simulink model "DSC4to1Diodes"  (R2022a)
settings: Solver=VariableStepAuto  StartTime=0.0  StopTime=10.0  RelTol=1e-3
undefined symbols (not defined in the file): plecs
settings Model: Creator=dcostine  LastModifiedBy=dcostine
settings DebuggingCC: UnconnectedInputMsg=warning  UnconnectedOutputMsg=warning  UnconnectedLineMsg=warning
settings RTWCC: DLArmComputeVersion=19.05

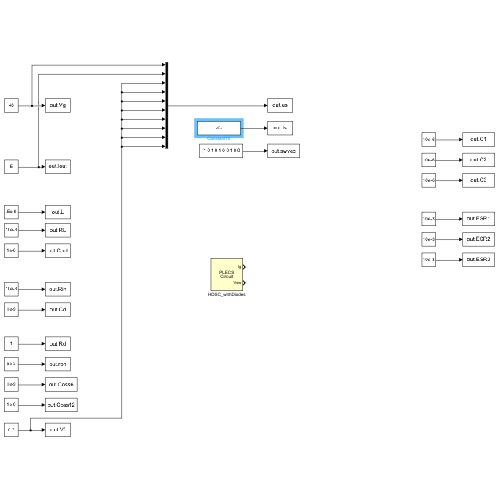
[thumbnail: Simulink's stored preview of the top-level diagram]
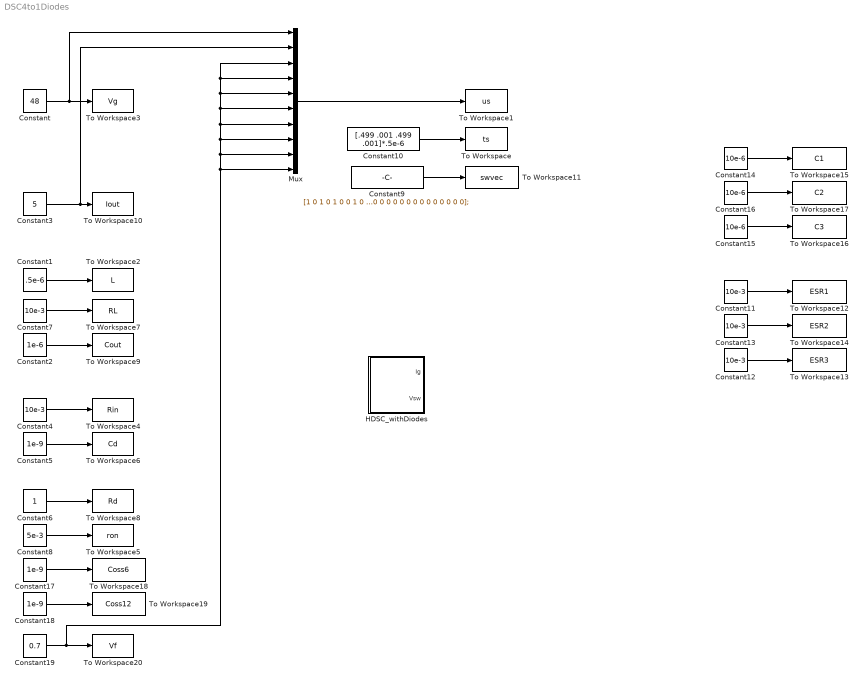
== system DSC4to1Diodes ==
  Constant : Constant  Value=48
  Constant1 : Constant  Value=.5e-6
  Constant10 : Constant  Value=[.499 .001 .499 .001]*.5e-6
  Constant{4,7,11..13} (5 alike) : Constant  Value=10e-3
  Constant14 : Constant  Value=10e-6
  Constant15 : Constant  Value=10e-6
  Constant16 : Constant  Value=10e-6
  Constant17 : Constant  Value=1e-9
  Constant18 : Constant  Value=1e-9
  Constant19 : Constant  Value=0.7
  Constant2 : Constant  Value=1e-6
  Constant3 : Constant  Value=5
  Constant5 : Constant  Value=1e-9
  Constant6 : Constant
  Constant8 : Constant  Value=5e-3
  Constant9 : Constant  Value=[1 0 1 0 1 0 0 1 0 0 0 0 0 0 0 0; 0 0 0 0 0 0 0 0 0 0 0 0 0 0 0 0; 0 1 0 1 0 1 1 0 0 0 0 0 0 0 0 0; 0 0 0 0 0 0 0 0 0 0 0 0 0 0 0 0];
  HDSC_withDiodes : Subsystem  LoadFcn=plecs('sl', 200);  InitFcn=plecs('sl', 214);  StartFcn=plecs('sl', 208);  StopFcn=plecs('sl', 209);  mask(PlecsCircuit){PLECSData=<binary blob, 3580 chars, not shown>}
      mask prompts: PLECSData "PLECS Data (Do not delete or modify!)"
      mask init:
      | % PLACE CUSTOM INITIALIZATIONS ABOVE
      | % DO NOT REMOVE
      | plecs('sl', 215);
      | % DO NOT REMOVE
      settings: CopyFcn=plecs('sl', 203);  DeleteFcn=plecs('sl', 205);  UndoDeleteFcn=plecs('sl', 206);  PreSaveFcn=plecs('sl', 211);  PostSaveFcn=plecs('sl', 201);  NameChangeFcn=plecs('sl', 210);  DestroyFcn=plecs('sl', 207);  PreCopyFcn=plecs('sl', 216);  OpenFcn=plecs('sl', 202);  ErrorFcn=plerrorfcn
      mask Help: web(['file:///' fullfile(plecsdoc, 'creatingacircuit.html')])
      mask Display: disp('PLECS\nCircuit')
  Mux : Mux  Inputs=10
  To Workspace : ToWorkspace  VariableName=ts  SampleTime=-1
  To Workspace1 : ToWorkspace  VariableName=us  SampleTime=-1
  To Workspace10 : ToWorkspace  VariableName=Iout  SampleTime=-1
  To Workspace11 : ToWorkspace  VariableName=swvec  SampleTime=-1
  To Workspace12 : ToWorkspace  VariableName=ESR1  SampleTime=-1
  To Workspace13 : ToWorkspace  VariableName=ESR3  SampleTime=-1
  To Workspace14 : ToWorkspace  VariableName=ESR2  SampleTime=-1
  To Workspace15 : ToWorkspace  VariableName=C1  SampleTime=-1
  To Workspace16 : ToWorkspace  VariableName=C3  SampleTime=-1
  To Workspace17 : ToWorkspace  VariableName=C2  SampleTime=-1
  To Workspace18 : ToWorkspace  VariableName=Coss6  SampleTime=-1
  To Workspace19 : ToWorkspace  VariableName=Coss12  SampleTime=-1
  To Workspace2 : ToWorkspace  VariableName=L  SampleTime=-1
  To Workspace20 : ToWorkspace  VariableName=Vf  SampleTime=-1
  To Workspace3 : ToWorkspace  VariableName=Vg  SampleTime=-1
  To Workspace4 : ToWorkspace  VariableName=Rin  SampleTime=-1
  To Workspace5 : ToWorkspace  VariableName=ron  SampleTime=-1
  To Workspace6 : ToWorkspace  VariableName=Cd  SampleTime=-1
  To Workspace7 : ToWorkspace  VariableName=RL  SampleTime=-1
  To Workspace8 : ToWorkspace  VariableName=Rd  SampleTime=-1
  To Workspace9 : ToWorkspace  VariableName=Cout  SampleTime=-1
  wires:
  Mux/1 -> To Workspace1/1
  Constant1/1 -> To Workspace2/1
  Constant/1 -> Mux/1, To Workspace3/1
  Constant9/1 -> To Workspace11/1
  Constant8/1 -> To Workspace5/1
  Constant2/1 -> To Workspace9/1
  Constant5/1 -> To Workspace6/1
  Constant3/1 -> Mux/2, To Workspace10/1
  Constant10/1 -> To Workspace/1
  Constant4/1 -> To Workspace4/1
  Constant11/1 -> To Workspace12/1
  Constant12/1 -> To Workspace13/1
  Constant13/1 -> To Workspace14/1
  Constant15/1 -> To Workspace16/1
  Constant16/1 -> To Workspace17/1
  Constant14/1 -> To Workspace15/1
  Constant17/1 -> To Workspace18/1
  Constant18/1 -> To Workspace19/1
  Constant7/1 -> To Workspace7/1
  Constant19/1 -> Mux/9, Mux/8, Mux/7, Mux/6, Mux/5, Mux/4, Mux/3, Mux/10, To Workspace20/1
  Constant6/1 -> To Workspace8/1

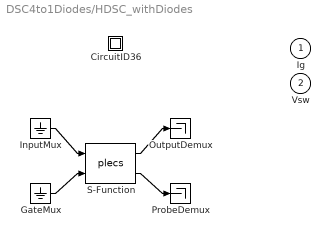
== system DSC4to1Diodes/HDSC_withDiodes ==
  " CircuitID36 " : Subsystem
  " GateMux " : Ground
  " InputMux " : Ground
  " OutputDemux " : Terminator
  " ProbeDemux " : Terminator
  " S-Function " : S-Function  FunctionName=plecs  SFunctionDeploymentMode=off  EnableBusSupport=off
  Ig : Outport  VectorParamsAs1DForOutWhenUnconnected=off
  Vsw : Outport  Port=2  VectorParamsAs1DForOutWhenUnconnected=off
  wires:
  " InputMux "/1 -> " S-Function "/1
  " GateMux "/1 -> " S-Function "/2
  " S-Function "/1 -> " OutputDemux "/1
  " S-Function "/2 -> " ProbeDemux "/1

== system DSC4to1Diodes/HDSC_withDiodes/ CircuitID36  ==
